simulink model "M2_TorqueDriven_Validation"  (R2025b)
settings: Solver=ode15s  StartTime=0.0  StopTime=T_stop  MaxStep=1e-3  RelTol=1e-8  AbsTol=1e-9  EnableMultiTasking=on
undefined symbols (not defined in the file): d4_A, d4_B, F0_y, I3_0, I4_0, Kd3, Kd4, Ki3, Ki4, Kp3, Kp4, omega_F, omega_traj, q3_A, q3_B, Ts_log, X, Y, Z
libraries: nesl_utility x12, sm_lib x9
Description:
  | MS02P08B torque-driven plant. Built 2026-11-18 13:07 by build_M2_TorqueDriven_Validation.m from M2_LoadInjection.slx (MD5 f17dcb99da107e28bae416fc79d4f5ec). Plant parameters: Rasuli 2014 Table II (Machine A). Do not edit by hand; rebuild.
settings Model: Creator=Mritunjoy Hazra  LastModifiedBy=IIT KGP
settings SolverCC: AutoScaleAbsTol=off  AlgebraicLoopSolver=TrustRegion  MaxZcPerStep=1.0
settings DataIOCC: LimitDataPoints=on  MaxDataPoints=10000  OutputTimes=0:0.01:30
settings OptimizationCC: ReuseModelBlockBuffer=off  LifeSpan=inf
settings DebuggingCC: UnconnectedInputMsg=warning  UnconnectedOutputMsg=warning  UnconnectedLineMsg=warning  AllowSymbolicDim=off  SubsystemReferenceDiagnosticForUnitTest=warning  SFUnexpectedBacktrackingDiag=warning  SFNoUnconditionalDefaultTransitionDiag=warning  SFExecutionAtInitializationDiag=none  ArithmeticOperatorsInVariantConditions=warning
settings ModelReferenceCC: EnableRefExpFcnMdlSchedulingChecks=on
settings SFSimCC: SimUseLocalCustomCode=off  CustomCodeUndefinedFunction=UseInterfaceOnly
settings RTWCC: RTWUseLocalCustomCode=off  GPUComputeCapability=3.5  DLArmComputeVersion=19.05
settings CodeAppCC: StateflowObjectComments=on
settings GRTTargetCC: TargetLangStandard=C89/C90 (ANSI)
settings ConfigComp: CovMetricSettings=dw  CovSaveCumulativeToWorkspaceVar=on  CovSaveSingleToWorkspaceVar=on  CovExternalEMLEnable=off  CovSFcnEnable=off
settings SimscapeCC: SimscapeLogType=all  SimscapeLogSimulationStatistics=on  SimscapeLogDataHistory=10000.0

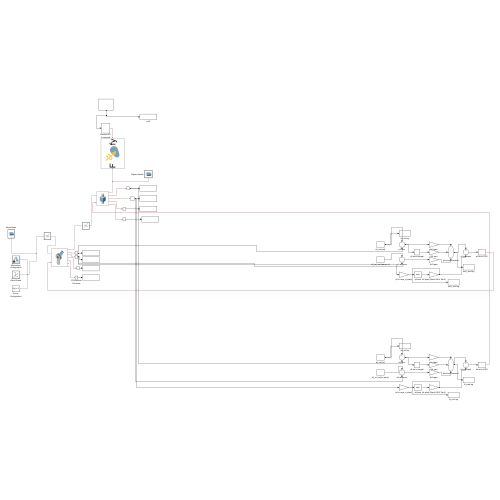
[thumbnail: Simulink's stored preview of the top-level diagram]
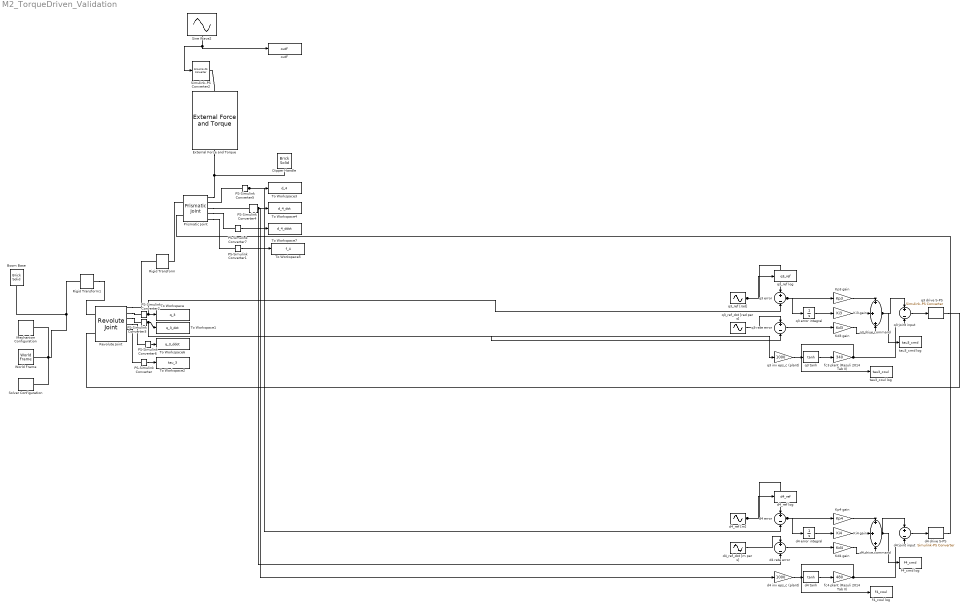
== system M2_TorqueDriven_Validation ==
  Boom Base : sm_lib/Body Elements/Brick Solid  BrickDimensions=[1 1 1]  BrickDimensionsUnits=m  ExportEntireGeometry=off  InertiaType=Custom  BasedOnType=Density  Density=1000  DensityUnits=kg/m^3  Mass=135000  MassUnits=kg  CenterOfMass=[8 0 0]  CenterOfMassUnits=m  MomentsOfInertia=[0 0 2500000]  MomentsOfInertiaUnits=kg*m^2  ProductsOfInertia=[0 0 0]  ProductsOfInertiaUnits=kg*m^2  GraphicType=FromGeometry  MarkerShape=Sphere  MarkerSize=10  GraphicVisPropType=SimpleVisualProperties  GraphicDiffuseColor=[0.5 0.5 0.5]  GraphicOpacity=1.0  GraphicSpecularColor=[0.5 0.5 0.5 1.0]  GraphicAmbientColor=[0.15 0.15 0.15 1.0]  GraphicEmissiveColor=[0.0 0.0 0.0 1.0]  GraphicShininess=75  DoExposeReferenceFrame=on  SerializedFrames=<Frames/>
  Dipper Handle : sm_lib/Body Elements/Brick Solid  BrickDimensions=[1 1 1]  BrickDimensionsUnits=m  ExportEntireGeometry=off  InertiaType=Custom  BasedOnType=Density  Density=1000  DensityUnits=kg/m^3  Mass=[54300]  MassUnits=kg  CenterOfMass=[0 0 -2.82]  CenterOfMassUnits=m  MomentsOfInertia=[287900 0 0 ]  MomentsOfInertiaUnits=kg*m^2  ProductsOfInertia=[0 0 0]  ProductsOfInertiaUnits=kg*m^2  GraphicType=FromGeometry  MarkerShape=Sphere  MarkerSize=10  GraphicVisPropType=SimpleVisualProperties  GraphicDiffuseColor=[0.5 0.5 0.5]  GraphicOpacity=1  GraphicSpecularColor=[0.5 0.5 0.5 1.0]  GraphicAmbientColor=[0.15 0.15 0.15 1.0]  GraphicEmissiveColor=[0.0 0.0 0.0 1.0]  GraphicShininess=75  DoExposeReferenceFrame=on  SerializedFrames=<Frames/>
  External Force and Torque : sm_lib/Forces and Torques/External Force and Torque  EnableForceX=off  EnableForceY=on  EnableForceZ=off  EnableForce=off  ForceResolutionFrame=World  EnableTorqueX=off  EnableTorqueY=off  EnableTorqueZ=off  EnableTorque=off  TorqueResolutionFrame=AttachedFrame
  Kd3 gain : Gain  Gain=Kd3
  Kd4 gain : Gain  Gain=Kd4
  Ki3 gain : Gain  Gain=Ki3
  Ki4 gain : Gain  Gain=Ki4
  Kp3 gain : Gain  Gain=Kp3
  Kp4 gain : Gain  Gain=Kp4
  Mechanism Configuration : sm_lib/Utilities/Mechanism Configuration  UniformGravity=Constant  GravityVector=[0 -9.80665 0]  GravityVectorUnits=m/s^2  LinearizationDelta=0.001  JointModeTransitionNonlinearIterations=2
  PS-Simulink Converter : nesl_utility/PS-Simulink Converter  PhysicalDomain=network_engine_domain  SubClassName=ps_output  LeftPortType=input  RightPortType=output  PseudoPeriodic=off  Frequencies=[]  VectorFormat=inherit  Unit=N*m  AffineConversion=off
  PS-Simulink Converter1 : nesl_utility/PS-Simulink Converter  PhysicalDomain=network_engine_domain  SubClassName=ps_output  LeftPortType=input  RightPortType=output  PseudoPeriodic=off  Frequencies=[]  VectorFormat=inherit  Unit=N  AffineConversion=off
  PS-Simulink Converter2 : nesl_utility/PS-Simulink Converter  PhysicalDomain=network_engine_domain  SubClassName=ps_output  LeftPortType=input  RightPortType=output  PseudoPeriodic=off  Frequencies=[]  VectorFormat=inherit  Unit=rad  AffineConversion=off
  PS-Simulink Converter3 : nesl_utility/PS-Simulink Converter  PhysicalDomain=network_engine_domain  SubClassName=ps_output  LeftPortType=input  RightPortType=output  PseudoPeriodic=off  Frequencies=[]  VectorFormat=inherit  Unit=rad/s  AffineConversion=off
  PS-Simulink Converter4 : nesl_utility/PS-Simulink Converter  PhysicalDomain=network_engine_domain  SubClassName=ps_output  LeftPortType=input  RightPortType=output  PseudoPeriodic=off  Frequencies=[]  VectorFormat=inherit  Unit=m/s  AffineConversion=off
  PS-Simulink Converter5 : nesl_utility/PS-Simulink Converter  PhysicalDomain=network_engine_domain  SubClassName=ps_output  LeftPortType=input  RightPortType=output  PseudoPeriodic=off  Frequencies=[]  VectorFormat=inherit  Unit=m  AffineConversion=off
  PS-Simulink Converter6 : nesl_utility/PS-Simulink Converter  PhysicalDomain=network_engine_domain  SubClassName=ps_output  LeftPortType=input  RightPortType=output  PseudoPeriodic=off  Frequencies=[]  VectorFormat=inherit  Unit=rad/s^2  AffineConversion=off
  PS-Simulink Converter7 : nesl_utility/PS-Simulink Converter  PhysicalDomain=network_engine_domain  SubClassName=ps_output  LeftPortType=input  RightPortType=output  PseudoPeriodic=off  Frequencies=[]  VectorFormat=inherit  Unit=m/s^2  AffineConversion=off
  Prismatic Joint : sm_lib/Joints/Prismatic Joint  JointMode=Normal  CompositeWrenchDir=FollowerOnBase  CompositeWrenchFrame=BaseFrame  SenseConstraintForce=off  SenseConstraintTorque=off  SenseTotalForce=off  SenseTotalTorque=off  PositionTargetSpecify=on  PositionTargetPriority=High  PositionTargetValue=d4_0  PositionTargetValueUnits=m  VelocityTargetSpecify=on  VelocityTargetPriority=High  VelocityTargetValue=d4d_0  VelocityTargetValueUnits=m/s  EquilibriumPosition=0  EquilibriumPositionUnits=m  SpringStiffness=0  SpringStiffnessUnits=N/m  DampingCoefficient=1473.0  DampingCoefficientUnits=N/(m/s)  LowerLimitSpecify=off  LowerLimitBound=-1  LowerLimitBoundUnits=m  LowerLimitStiffness=1e6  LowerLimitStiffnessUnits=N/m  LowerLimitDamping=1e3  LowerLimitDampingUnits=N/(m/s)  LowerLimitTransitionRegionWidth=1e-4  LowerLimitTransitionRegionWidthUnits=m  UpperLimitSpecify=off  UpperLimitBound=1  UpperLimitBoundUnits=m  UpperLimitStiffness=1e6  UpperLimitStiffnessUnits=N/m  UpperLimitDamping=1e3  UpperLimitDampingUnits=N/(m/s)  UpperLimitTransitionRegionWidth=1e-4  UpperLimitTransitionRegionWidthUnits=m  TorqueActuationMode=InputTorque  MotionActuationMode=ComputedMotion  SensePosition=on  SenseVelocity=on  SenseAcceleration=on  SenseTorqueForce=on  SenseLowerLimitTorqueForce=off  SenseUpperLimitTorqueForce=off
  Revolute Joint : sm_lib/Joints/Revolute Joint  JointMode=Normal  CompositeWrenchDir=FollowerOnBase  CompositeWrenchFrame=BaseFrame  SenseConstraintForce=off  SenseConstraintTorque=off  SenseTotalForce=on  SenseTotalTorque=on  PositionTargetSpecify=on  PositionTargetPriority=High  PositionTargetValue=q3_0_deg  PositionTargetValueUnits=deg  VelocityTargetSpecify=on  VelocityTargetPriority=High  VelocityTargetValue=q3d_0_degps  VelocityTargetValueUnits=deg/s  EquilibriumPosition=0  EquilibriumPositionUnits=deg  SpringStiffness=0  SpringStiffnessUnits=N*m/deg  DampingCoefficient=66.322512  DampingCoefficientUnits=N*m/(deg/s)  LowerLimitSpecify=off  LowerLimitBound=-90  LowerLimitBoundUnits=deg  LowerLimitStiffness=1e4  LowerLimitStiffnessUnits=N*m/deg  LowerLimitDamping=10  LowerLimitDampingUnits=N*m/(deg/s)  LowerLimitTransitionRegionWidth=0.1  LowerLimitTransitionRegionWidthUnits=deg  UpperLimitSpecify=off  UpperLimitBound=90  UpperLimitBoundUnits=deg  UpperLimitStiffness=1e4  UpperLimitStiffnessUnits=N*m/deg  UpperLimitDamping=10  UpperLimitDampingUnits=N*m/(deg/s)  UpperLimitTransitionRegionWidth=0.1  UpperLimitTransitionRegionWidthUnits=deg  TorqueActuationMode=InputTorque  MotionActuationMode=ComputedMotion  SensePosition=on  SenseVelocity=on  SenseAcceleration=on  SenseTorqueForce=on  SenseLowerLimitTorqueForce=off  SenseUpperLimitTorqueForce=off
  Rigid Transform : sm_lib/Frames and Transforms/Rigid Transform  RotationMethod=StandardAxis  FollAlignAxisA=+X  BaseAlignAxisA=+Y  FollAlignAxisB=+Y  BaseAlignAxisB=+Z  RotationStandardAxis=+Y  RotationAngle=90  RotationAngleUnits=deg  RotationArbitraryAxis=[0 0 1]  RotationSequenceAxes=FollowerAxes  RotationSequence=XYX  RotationSequenceAngles=[0 0 0]  RotationSequenceAnglesUnits=deg  RotationMatrix=[1 0 0;0 1 0;0 0 1]  Quaternion=[1 0 0 0]  TranslationMethod=Cartesian  TranslationCartesianOffset=[1.5 0 0]  TranslationCartesianOffsetUnits=m  TranslationStandardAxis=+Z  TranslationStandardOffset=0  TranslationStandardOffsetUnits=m  TranslationROffset=0  TranslationROffsetUnits=m  TranslationThetaOffset=0  TranslationThetaOffsetUnits=deg  TranslationZOffset=0  TranslationZOffsetUnits=m
  Rigid Transform1 : sm_lib/Frames and Transforms/Rigid Transform  RotationMethod=None  FollAlignAxisA=+X  BaseAlignAxisA=+Y  FollAlignAxisB=+Y  BaseAlignAxisB=+Z  RotationStandardAxis=+X  RotationAngle=90  RotationAngleUnits=deg  RotationArbitraryAxis=[0 0 1]  RotationSequenceAxes=FollowerAxes  RotationSequence=XYX  RotationSequenceAngles=[0 0 0]  RotationSequenceAnglesUnits=deg  RotationMatrix=[1 0 0;0 1 0;0 0 1]  Quaternion=[1 0 0 0]  TranslationMethod=Cartesian  TranslationCartesianOffset=[0 0 0]  TranslationCartesianOffsetUnits=m  TranslationStandardAxis=+Z  TranslationStandardOffset=0  TranslationStandardOffsetUnits=m  TranslationROffset=0  TranslationROffsetUnits=m  TranslationThetaOffset=0  TranslationThetaOffsetUnits=deg  TranslationZOffset=0  TranslationZOffsetUnits=m
  Simulink-PS Converter2 : nesl_utility/Simulink-PS Converter  PhysicalDomain=network_engine_domain  SubClassName=ps_input  LeftPortType=input  RightPortType=output  PseudoPeriodic=off  Frequencies=[]  NoiseDistribution=none  NoiseParameters=[]  Unit=N  AffineConversion=off  FilteringAndDerivatives=zero  SimscapeFilterOrder=2  InputFilterTimeConstant=0.05  UdotUserProvided=0
  Sine Wave2 : Sin  Amplitude=F0_y  Frequency=omega_F  SampleTime=0
  Solver Configuration : nesl_utility/Solver Configuration  PhysicalDomain=network_engine_domain  SubClassName=solver  LeftPortType=input  RightPortType=generic  Tones=[]  Harmonics=[]  SimulateNoise=off  Profile=off  UseLocalSampling=off  EnableSwitchedLinearOptims=on  FrequencyDomain=off  UseCCode=off  RelTol=0.001  AbsTol=1e-06  MinStep=1e-09  ToWorkspace=off  RevertToSquareIcSolve=off  NumHomotopyIterations=100  PhasorMode=off  PhasorModeNumHarmonics=1  ConsistencySolver=NEWTON_XTOL_AFTER_FTOL  IndexReductionMethod=DerivativeReplacement  DoDC=off  ResidualTolerance=1e-09  ConsistencyTolSource=GLOBAL  ConsistencyAbsTol=0.001  ConsistencyRelTol=0.001  ConsistencyTolFactor=0.001  UseLocalSolver=off  LocalSolverChoice=NE_BACKWARD_EULER_ADVANCER  ResolveIndetEquations=on  FunctionEvalNumThread=1  LocalSolverSampleTime=0.001  DoFixedCost=off  MaxNonlinIter=3  MaxModeIter=2  ComputeImpulses=off  ImpulseIterations=2  LinearAlgebra=Sparse  LinearAlgebraNumThread=0  EquationFormulation=NE_TIME_EF  DelaysMemoryBudget=1024  AutomaticFiltering=on  FilteringTimeConstant=0.001  PartitionStorageMethod=AS_NEEDED  PartitionMemoryBudget=1024  PartitionMethod=FAST  MultibodyUseLocalSolver=off  MultibodyLocalSolverChoice=ODE1  MultibodyLocalSolverSampleTime=0.001
  To Workspace : ToWorkspace  VariableName=q_3  SaveFormat=Timeseries  SampleTime=Ts_log
  To Workspace1 : ToWorkspace  VariableName=q_3_dot  SaveFormat=Timeseries  SampleTime=Ts_log
  To Workspace2 : ToWorkspace  VariableName=tau_3  SaveFormat=Timeseries  SampleTime=Ts_log
  To Workspace3 : ToWorkspace  VariableName=d_4  SaveFormat=Timeseries  SampleTime=Ts_log
  To Workspace4 : ToWorkspace  VariableName=d_4_dot  SaveFormat=Timeseries  SampleTime=Ts_log
  To Workspace5 : ToWorkspace  VariableName=f_4  SaveFormat=Timeseries  SampleTime=Ts_log
  To Workspace6 : ToWorkspace  VariableName=q_3_ddot  SaveFormat=Timeseries  SampleTime=Ts_log
  To Workspace7 : ToWorkspace  VariableName=d_4_ddot  SaveFormat=Timeseries  SampleTime=Ts_log
  World Frame : sm_lib/Frames and Transforms/World Frame
  d4 drive S-PS : nesl_utility/Simulink-PS Converter  PhysicalDomain=network_engine_domain  SubClassName=ps_input  LeftPortType=input  RightPortType=output  PseudoPeriodic=off  Frequencies=[]  NoiseDistribution=none  NoiseParameters=[]  Unit=N  AffineConversion=off  FilteringAndDerivatives=zero  SimscapeFilterOrder=2  InputFilterTimeConstant=0.05  UdotUserProvided=0
  d4 drive command : Sum  Inputs=+++
  d4 error : Sum  Inputs=+-
  d4 error integral : Integrator  InitialCondition=I4_0
  d4 inv eps_c (plant) : Gain  Gain=1000
  d4 joint input : Sum  Inputs=+-
  d4 rate error : Sum  Inputs=+-
  d4 tanh : Trigonometry  Operator=tanh
  d4_ref [m] : Sin  Amplitude=d4_A  Bias=d4_B  Frequency=omega_traj  SampleTime=0
  d4_ref log : ToWorkspace  VariableName=d4_ref  SaveFormat=Timeseries  SampleTime=Ts_log
  d4_ref_dot [m per s] : Sin  Amplitude=d4_A*omega_traj  Frequency=omega_traj  Phase=pi/2  SampleTime=0
  f4_cmd log : ToWorkspace  VariableName=f4_cmd  SaveFormat=Timeseries  SampleTime=Ts_log
  f4_coul log : ToWorkspace  VariableName=f4_coul  SaveFormat=Timeseries  SampleTime=Ts_log
  fc3 plant (Rasuli 2014 Tab II) : Gain  Gain=340
  fc4 plant (Rasuli 2014 Tab II) : Gain  Gain=480
  outF : ToWorkspace  VariableName=outF  SaveFormat=Timeseries  SampleTime=Ts_log
  q3 drive S-PS : nesl_utility/Simulink-PS Converter  PhysicalDomain=network_engine_domain  SubClassName=ps_input  LeftPortType=input  RightPortType=output  PseudoPeriodic=off  Frequencies=[]  NoiseDistribution=none  NoiseParameters=[]  Unit=N*m  AffineConversion=off  FilteringAndDerivatives=zero  SimscapeFilterOrder=2  InputFilterTimeConstant=0.05  UdotUserProvided=0
  q3 drive command : Sum  Inputs=+++
  q3 error : Sum  Inputs=+-
  q3 error integral : Integrator  InitialCondition=I3_0
  q3 inv eps_c (plant) : Gain  Gain=1000
  q3 joint input : Sum  Inputs=+-
  q3 rate error : Sum  Inputs=+-
  q3 tanh : Trigonometry  Operator=tanh
  q3_ref [rad] : Sin  Amplitude=q3_A  Bias=q3_B  Frequency=omega_traj  SampleTime=0
  q3_ref log : ToWorkspace  VariableName=q3_ref  SaveFormat=Timeseries  SampleTime=Ts_log
  q3_ref_dot [rad per s] : Sin  Amplitude=q3_A*omega_traj  Frequency=omega_traj  Phase=pi/2  SampleTime=0
  tau3_cmd log : ToWorkspace  VariableName=tau3_cmd  SaveFormat=Timeseries  SampleTime=Ts_log
  tau3_coul log : ToWorkspace  VariableName=tau3_coul  SaveFormat=Timeseries  SampleTime=Ts_log
  wires:
  PS-Simulink Converter1/1 -> To Workspace5/1
  PS-Simulink Converter2/1 -> To Workspace/1, q3 error/2
  PS-Simulink Converter3/1 -> To Workspace1/1, q3 rate error/2, q3 inv eps_c (plant)/1
  PS-Simulink Converter/1 -> To Workspace2/1
  PS-Simulink Converter4/1 -> To Workspace4/1, d4 rate error/2, d4 inv eps_c (plant)/1
  PS-Simulink Converter5/1 -> To Workspace3/1, d4 error/2
  PS-Simulink Converter6/1 -> To Workspace6/1
  PS-Simulink Converter7/1 -> To Workspace7/1
  Sine Wave2/1 -> Simulink-PS Converter2/1, outF/1
  q3_ref [rad]/1 -> q3 error/1, q3_ref log/1
  q3_ref_dot [rad per s]/1 -> q3 rate error/1
  q3 error/1 -> Kp3 gain/1, q3 error integral/1
  q3 error integral/1 -> Ki3 gain/1
  q3 rate error/1 -> Kd3 gain/1
  Kp3 gain/1 -> q3 drive command/1
  Ki3 gain/1 -> q3 drive command/2
  Kd3 gain/1 -> q3 drive command/3
  q3 inv eps_c (plant)/1 -> q3 tanh/1
  q3 tanh/1 -> fc3 plant (Rasuli 2014 Tab II)/1
  q3 drive command/1 -> q3 joint input/1, tau3_cmd log/1
  fc3 plant (Rasuli 2014 Tab II)/1 -> q3 joint input/2, tau3_coul log/1
  q3 joint input/1 -> q3 drive S-PS/1
  d4_ref [m]/1 -> d4 error/1, d4_ref log/1
  d4_ref_dot [m per s]/1 -> d4 rate error/1
  d4 error/1 -> Kp4 gain/1, d4 error integral/1
  d4 error integral/1 -> Ki4 gain/1
  d4 rate error/1 -> Kd4 gain/1
  Kp4 gain/1 -> d4 drive command/1
  Ki4 gain/1 -> d4 drive command/2
  Kd4 gain/1 -> d4 drive command/3
  d4 inv eps_c (plant)/1 -> d4 tanh/1
  d4 tanh/1 -> fc4 plant (Rasuli 2014 Tab II)/1
  d4 drive command/1 -> d4 joint input/1, f4_cmd log/1
  fc4 plant (Rasuli 2014 Tab II)/1 -> d4 joint input/2, f4_coul log/1
  d4 joint input/1 -> d4 drive S-PS/1
  connections:
  Boom Base/RConn1 -- Rigid Transform1/LConn1 -- Solver Configuration/RConn1 -- World Frame/RConn1 -- Mechanism Configuration/RConn1
  Revolute Joint/RConn5 -- PS-Simulink Converter/LConn1
  Revolute Joint/RConn1 -- Rigid Transform/LConn1
  Rigid Transform/RConn1 -- Prismatic Joint/LConn1
  Prismatic Joint/RConn1 -- External Force and Torque/RConn1 -- Dipper Handle/RConn1
  Revolute Joint/RConn2 -- PS-Simulink Converter2/LConn1
  Revolute Joint/RConn3 -- PS-Simulink Converter3/LConn1
  Prismatic Joint/RConn5 -- PS-Simulink Converter1/LConn1
  Prismatic Joint/RConn3 -- PS-Simulink Converter4/LConn1
  PS-Simulink Converter5/LConn1 -- Prismatic Joint/RConn2
  Rigid Transform1/RConn1 -- Revolute Joint/LConn1
  Revolute Joint/RConn4 -- PS-Simulink Converter6/LConn1
  Prismatic Joint/RConn4 -- PS-Simulink Converter7/LConn1
  External Force and Torque/LConn1 -- Simulink-PS Converter2/RConn1
  q3 drive S-PS/RConn1 -- Revolute Joint/LConn2
  d4 drive S-PS/RConn1 -- Prismatic Joint/LConn2
